simulink model "Valley_FiuPFC"  (R2023b)
settings: Solver=VariableStepAuto  StartTime=0.0  StopTime=0.5  RelTol=1e-3
libraries: spsDiodeLib x11, spsSeriesRLCBranchLib x5, spsACVoltageSourceLib x2, spsCurrentMeasurementLib x2, spsVoltageMeasurementLib x2, sps_lib x1
settings Model: Creator=yigex  LastModifiedBy=yigex

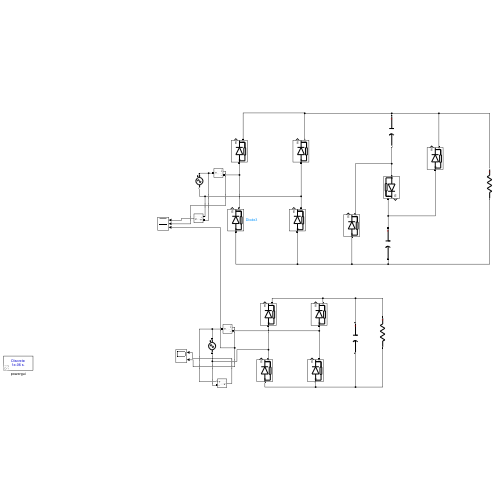
[thumbnail: Simulink's stored preview of the top-level diagram]
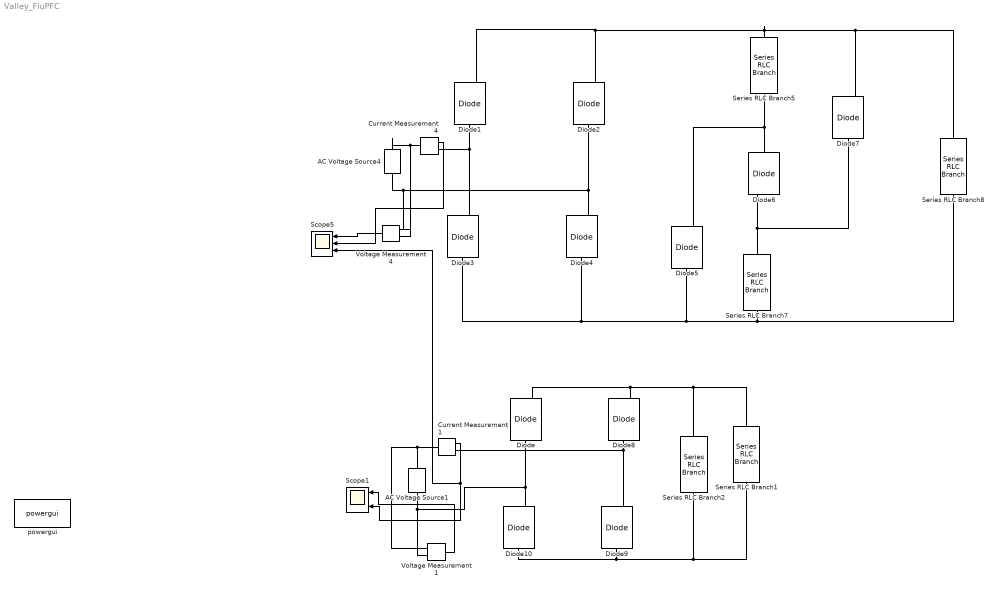
== system Valley_FiuPFC ==
  AC Voltage Source1 : spsACVoltageSourceLib/AC Voltage Source  Amplitude=310  Phase=0  Frequency=60  SampleTime=0  Measurements=None  BusType=swing  Pref=10e3  Qref=0  Qmin=-inf  Qmax=+inf
  AC Voltage Source4 : spsACVoltageSourceLib/AC Voltage Source  Amplitude=310  Phase=0  Frequency=60  SampleTime=0  Measurements=None  BusType=swing  Pref=10e3  Qref=0  Qmin=-inf  Qmax=+inf
  Current Measurement1 : spsCurrentMeasurementLib/Current Measurement  PhasorSimulation=off  OutputType=Complex  PSBequivalent=0
  Current Measurement4 : spsCurrentMeasurementLib/Current Measurement  PhasorSimulation=off  OutputType=Complex  PSBequivalent=0
  Diode{,1..10} (11 alike) : spsDiodeLib/Diode  Ron=0.001  Lon=0  Vf=0.8  IC=0  UseSnubber=0  Rs=500  Cs=250e-9  Measurements=on
  Scope1 : Scope  NumInputPorts=2
  Scope5 : Scope  NumInputPorts=3
  Series RLC Branch1 : spsSeriesRLCBranchLib/Series RLC Branch  LConnTagsString=__new0  RConnTagsString=__new0  BranchType=R  Resistance=20  Inductance=220e-3  SetiL0=off  InitialCurrent=0  Capacitance=220e-6  Setx0=off  InitialVoltage=0  Measurements=None
  Series RLC Branch2 : spsSeriesRLCBranchLib/Series RLC Branch  LConnTagsString=__new0  RConnTagsString=__new0  BranchType=C  Resistance=10  Inductance=220e-3  SetiL0=off  InitialCurrent=0  Capacitance=220e-6  Setx0=off  InitialVoltage=0  Measurements=None
  Series RLC Branch5 : spsSeriesRLCBranchLib/Series RLC Branch  LConnTagsString=__new0  RConnTagsString=__new0  BranchType=C  Resistance=1  Inductance=220e-3  SetiL0=off  InitialCurrent=0  Capacitance=220e-6  Setx0=off  InitialVoltage=0  Measurements=None
  Series RLC Branch7 : spsSeriesRLCBranchLib/Series RLC Branch  LConnTagsString=__new0  RConnTagsString=__new0  BranchType=C  Resistance=1  Inductance=220e-3  SetiL0=off  InitialCurrent=0  Capacitance=220e-6  Setx0=off  InitialVoltage=0  Measurements=None
  Series RLC Branch8 : spsSeriesRLCBranchLib/Series RLC Branch  LConnTagsString=__new0  RConnTagsString=__new0  BranchType=R  Resistance=20  Inductance=1e-3  SetiL0=off  InitialCurrent=0  Capacitance=1e-6  Setx0=off  InitialVoltage=0  Measurements=None
  Voltage Measurement1 : spsVoltageMeasurementLib/Voltage Measurement  PhasorSimulation=off  OutputType=Complex  PSBequivalent=0
  Voltage Measurement4 : spsVoltageMeasurementLib/Voltage Measurement  PhasorSimulation=off  OutputType=Complex  PSBequivalent=0
  powergui : sps_lib/powergui  Priority=1  SimulationMode=Discrete  SampleTime=1e-6  frequency=60  Iterations=50  frequencyindice=60  Pbase=100e6  ErrMax=1e-4  UnitsV=kV  UnitsW=MW  buscounter=0  FunctionMessages=off  echomessages=off  EnableUseOfTLC=off  CurrentSourceSwitches=off  DisableSnubberDevices=off  DisableRonSwitches=off  DisableVfSwitches=off  DisplayEquations=off  AutomaticDiscreteSolvers=off  SolverType=Tustin/Backward Euler (TBE)  Interpol=off  ExternalGateDelay=off  methode=off  Ts=100  x0status=blocks  SPID=on  SwTol=0  HookPort=off  NonlinearTolerance=1e-4  nMaxIteration=100  ContinueOnMaxIteration=off  RestoreLinks=warning  ResistiveCurrentMeasurement=off  Frange=[0:2:500]  Ylog=off  Xlog=on  ShowGrid=off  save=off  variable=ZData  structure=0  ZoomFFT=off  StartTime=0.0  cycles=1  DisplayStyle=1  fundamental=60  FreqAxis=off  MaxFrequency=1000  frequencyindicesteady=1  RmsSteady=1  display=off
  wires:
  Voltage Measurement4/1 -> Scope5/1
  Current Measurement4/1 -> Scope5/2
  Voltage Measurement1/1 -> Scope1/1
  Current Measurement1/1 -> Scope5/3, Scope1/2
  connections:
  Diode3/RConn1 -- Current Measurement4/RConn1 -- Diode1/LConn1
  Diode4/RConn1 -- Voltage Measurement4/LConn2 -- AC Voltage Source4/LConn1 -- Diode2/LConn1
  Diode1/RConn1 -- Series RLC Branch5/LConn1 -- Diode7/RConn1 -- Series RLC Branch8/LConn1 -- Diode2/RConn1
  Diode3/LConn1 -- Series RLC Branch8/RConn1 -- Series RLC Branch7/RConn1 -- Diode5/LConn1 -- Diode4/LConn1
  Diode6/LConn1 -- Diode5/RConn1 -- Series RLC Branch5/RConn1
  Series RLC Branch7/LConn1 -- Diode7/LConn1 -- Diode6/RConn1
  AC Voltage Source4/RConn1 -- Voltage Measurement4/LConn1 -- Current Measurement4/LConn1
  Current Measurement1/LConn1 -- AC Voltage Source1/RConn1 -- Voltage Measurement1/LConn1
  Diode/LConn1 -- Diode10/RConn1 -- AC Voltage Source1/LConn1 -- Voltage Measurement1/LConn2
  Series RLC Branch1/RConn1 -- Diode10/LConn1 -- Diode9/LConn1 -- Series RLC Branch2/RConn1
  Diode8/LConn1 -- Diode9/RConn1 -- Current Measurement1/RConn1
  Diode8/RConn1 -- Diode/RConn1 -- Series RLC Branch2/LConn1 -- Series RLC Branch1/LConn1
